simulink model "BLDCSpeedControl_EV_Layout_FINAL"  (R2024b)
settings: Solver=ode23t  StartTime=0.0  StopTime=t_stop  FixedStep=Ts  MaxStep=5e-4  RelTol=1e-3  EnableMultiTasking=on
PreLoadFcn:
  | BLDCSpeedControlData;
values from neighbouring files (symbols this model uses):
  m = app.Rows(1:app.N, 1) >= 0.9*t    [EV_BlackBox_App.m]
  N = 0    [EV_BlackBox_App.m]
  p = inputParser    [Create_Simulation.m]    (also in EV_BlackBox_App.m = uipanel(parent, 'Title', title); Run_Simulation_Live.m; Run_Simulation_Log.m)
  s = regexprep(msg, '\s+', ' ')    [EV_BlackBox_App.m]    (also in Run_Simulation_Log.m = T.SOC(isfinite(T.SOC)))
undefined symbols (not defined in the file or in its folder): battery_builder_rtmsupport, cells_parallel, cells_series, DiscIntNeverNeededParam, Emax, Emax_thr, emf_max_ev, gcbh, I_cont, I_peak, Ke_ph, Kii, Kiv, Kiw, Kpi, Kpv, Kpw, load_scale, r_wheel, rpm_ramp, rpm_ref, T_Ifilt, Ts, Tsc, Vdc, Vlim_min, wheel_mass
libraries: nesl_utility x19, fl_lib x13, ee_lib x6, sm_lib x3, eeDiscretePi x2, Batteries2_lib x1, SignalEditorBlockLib x1, eePwmGenerator x1, eeGeneralControl x1
(part 1 of 2)
CloseFcn:
  | try,close(h1_BLDCSpeedControl),end
  | clear h1_BLDCSpeedControl
  | 
  | clear simlog_BLDCSpeedControl
  | clear logsout_BLDCSpeedControl
Description:
  | BLDC Speed Control
settings Model: Creator=The MathWorks, Inc.  LastModifiedBy=shubh
settings SolverCC: AlgebraicLoopSolver=TrustRegion  MaxZcPerStep=1
settings DataIOCC: MaxDataPoints=210000  ReturnWorkspaceOutputs=off  SignalLoggingName=logsout_BLDCSpeedControl
settings OptimizationCC: ReuseModelBlockBuffer=off  LifeSpan=inf
settings DebuggingCC: UnconnectedInputMsg=warning  UnconnectedOutputMsg=warning  UnconnectedLineMsg=warning  SFUnexpectedBacktrackingDiag=warning  SFNoUnconditionalDefaultTransitionDiag=warning  SFExecutionAtInitializationDiag=none  ArithmeticOperatorsInVariantConditions=warning
settings ModelReferenceCC: EnableRefExpFcnMdlSchedulingChecks=on
settings SFSimCC: SimUseLocalCustomCode=off  CustomCodeUndefinedFunction=UseInterfaceOnly
settings RTWCC: RTWUseLocalCustomCode=off  GPUComputeCapability=3.5  DLArmComputeVersion=19.05
settings CodeAppCC: StateflowObjectComments=on
settings GRTTargetCC: TargetLangStandard=C89/C90 (ANSI)
settings ConfigComp: CovMetricSettings=dw  CovSaveCumulativeToWorkspaceVar=on  CovSaveSingleToWorkspaceVar=on  CovExternalEMLEnable=off
settings SimscapeCC: SimscapeNormalizeSystem=off  SimscapeLogSimulationStatistics=on  SimscapeLogName=simlog_BLDCSpeedControl  SimscapeLogLimitData=off  SimscapeLogDataHistory=210000
settings ExplorerConfigSet: SimMechanicsOpenEditorOnUpdate=off

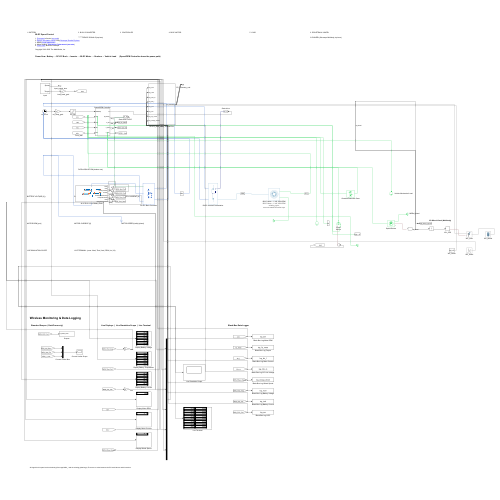
[thumbnail: Simulink's stored preview of the top-level diagram]
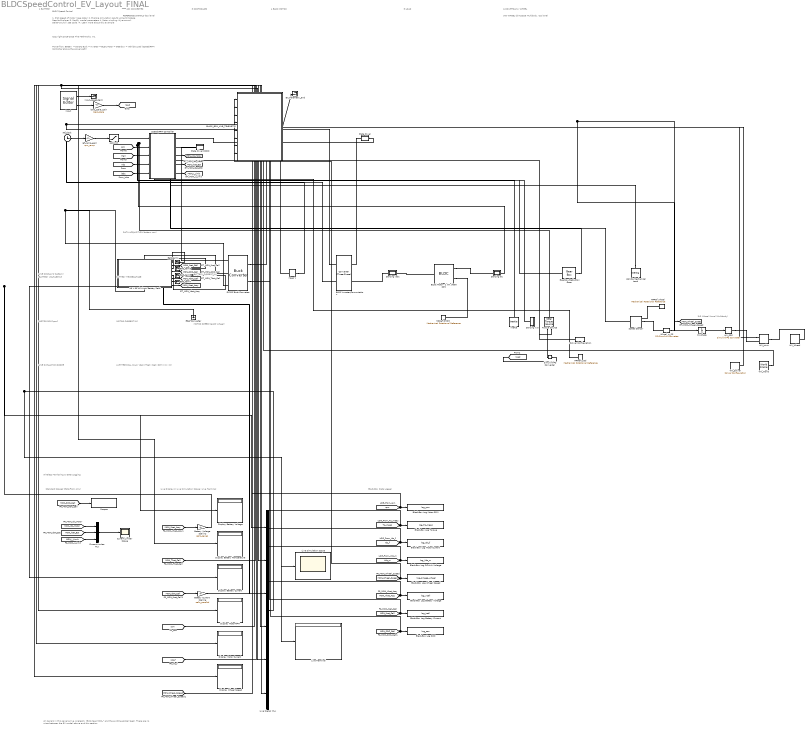
== system BLDCSpeedControl_EV_Layout_FINAL ==
  note: BLDC Speed Control
  note: 1. Plot speed of motor ( see code )
      | 2. Explore simulation results using Simscape Results Explorer
      | 3. Modify model parameters
      | 4. Motor winding: Wye-wound , Delta-wound ( see code )
      | 4. Learn more about this example
  note: Copyright 2016-2023 The MathWorks, Inc.
  note: BATTERY VOLTAGE [V]
  note: BATTERY TEMPERATURE
  note: BATTERY CURRENT [A]
  note: MOTOR RPM [rpm]
  note: MOTOR CURRENT [A]
  note: MOTOR SPEED [rad/s] (wheel)
  note: LIVE SIMULATION SCOPE
  note: LIVE TERMINAL (rows: Vbat | Tbat | Ibat | RPM | Im | W)
  note: 1 BATTERY
  note: 2 BUCK CONVERTER
  note: 3 CONTROLLER
  note: 4 BLDC MOTOR
  note: 5 LOAD
  note: 6 DRIVETRAIN / WHEEL
  note: REFERENCE SIGNALS (top lane)
  note: 3-D WHEEL (Simscape Multibody, top lane)
  note: DATA ACQUISITION (bottom row)
  note: LIVE DISPLAYS (bottom)
  note: Wireless Monitoring & Data Logging
  note: Standard Scopes (Goto/From only)
  note: Live Displays | Live Simulation Scope | Live Terminal
  note: Black-Box Data Logger
  note: All signals in this panel arrive wirelessly (Goto tags MON_* and the existing global tags). There are no wires between the EV model above and this section.
  note: Power flow: Battery → DC-DC Buck → Inverter → BLDC Motor → Gearbox → Vehicle Load (Speed/RPM Controller above the power path)
  note: 3-D Wheel Visual (Multibody)
  48 V 50 Ah Li-Ion Battery Pack : Subsystem  LoadFcn=battery_builder_rtmsupport('loadfcn',gcbh);
      settings: CopyFcn=battery_builder_rtmsupport('copyfcn',gcbh);  PreCopyFcn=battery_builder_rtmsupport('precopyfcn',gcbh);  PreDeleteFcn=battery_builder_rtmsupport('predeletefcn',gcbh);  PortSchema="{\"entries\":[{\"content\":{\"sides\":[{\"content\":{\"connectorIds\":[\"LConn1\"]},\"type\":\"ConnectorPlacement.EquallySpacedRectSide\",\"uuid\":\"bf691570-7ac9-499a-8942-6e8ffe2774e2\"},{\"content\":{\"connectorIds\":[\"RConn1\"],\"side\":\"RIGHT\"},\"type\":\"ConnectorPlacement.EquallySpacedRectSide\",\"uuid\":\"48e96f6a-2aee-45a9-a2ae-5a9441790c71\"},{\"content\":{\"side\":\"TOP\"},\"type\":\"ConnectorPlacement.EquallySpacedRectSide\",\"uuid\":\"dfdf2b0d-1e4b-464b-8a83-b0b25904b005\"},{\"content\":{\"connectorIds\":[\"Out1\",\"Out2\",\"Out3\",\"Out4\",\"Out5\",\"Out6\",\"Out7\",\"Out8\"],\"side\":\"BOTTOM\"},\"type\":\"ConnectorPlacement.EquallySpacedRectSide\",\"uuid\":\"0118fead-b379-4450-9723-57bbd90a7e7a\"}]},\"type\":\"ConnectorPlacement.EquallySpacedConnector\",\"uuid\":\"e9cae3f7-6351-471c-9be2-cb3ea8e3ac6a\"}],\"packageUris\":[\"http://schema.mathworks.com/mf0/Connector/R2020b\"],\"version\":\"1.0\"}"
      mask Display: image('$imagefile')
  BLACK_BOX_LIVE_TELEMETRY : Subsystem
  BLDC Inverter/Commutation : ee_lib/Semiconductors & Converters/Converters/Converter (Three-Phase)  port_option=ee.enum.threePhasePort.composite  fidelity_option=ee.enum.converters.fidelity.detailed  device_type=3  showThermalPort=false  K=0  Vth=0.5 V  Vgt=1 V  Vgt_off=-1 V  Ih=1 A  Vf=0.8 V  Ron=0.001 Ohm  Rds=0.001 Ohm  Goff=1e-5 1/Ohm  Eon_scalar=22.86e-3 J  Eoff_scalar=17.14e-3 J  Eoff_natural_commutation=10e-3 J  Voff=300 V  Iout_scalar=600 A  onCurrentMeasDelay=0 s  useCurrentFromPreviousCycle=false  useVoltageFromPreviousCycle=false  diode_param=2  diode_Vf=0.8 V  diode_Ron=0.001 Ohm  diode_Goff=1e-5 1/Ohm  diode_C=50 nF  diode_iRM=-235 A  diode_iF=300 A  diode_idot=-50 A/us  diode_trr_param=1  diode_trr_factor=3  diode_trr=15 us  diode_Qrr=1.5e+3 s*uA  diode_rec_loss_model=ee.enum.diode.reverseRecoveryModel.fixed  diode_ErecVal=0 J  diode_scaleWithIandV=false  diode_ErecMat=zeros(2, 3) J  diode_TjrecVec=[298.15, 398.15] K  diode_IfrecVec=[.1, 1, 10] A  diode_IrecVal=10 A  diode_VrecVal=10 V  diode_tFilter=1 / 1000 / 100 s  thermal_network_parameterization=ee.enum.thermalNetworkTopology.external  Rth=[.08, .5] K/W  Rth_Cauer=[.08, .1, .5] K/W  Rth_Foster=[.08, .14, .22, .16] K/W  thermal_mass_parameterization=ee.enum.thermalNetwork.timeconstant  thermal_mass=[.01, .5] J/K  thermal_mass_Cauer=[.01, .1, .5] J/K  thermal_mass_Foster=[.001, .005, .05, .5] J/K  thermal_time_constant=[.001, .2] s  thermal_time_constant_Cauer=[.001, .1, .2] s  thermal_time_constant_Foster=[7e-05, .0007, .01, .08] s  thermal_mass_initial_temperatures=[25, 25] degC  thermal_mass_initial_temperatures_Cauer=[25, 25, 25] degC  junction_thermal_mass=0.01 J/K  Tvec_initial_Foster=[25, 25, 25, 25] degC  snubber_type=0  Cs=1e-7 F  Rs=0.1 Ohm  Vce_loss=[0, 150, 300] V
  "BLDC Motor – 1 kW, 3000 RPM" : ee_lib/Electromechanical/Permanent Magnet/BLDC  port_option=ee.enum.threePhasePort.composite  rotor_param=1  pm_flux_linkage=psim Wb  theta_constant=pi / (2*p) rad  emf_max=emf_max_ev V  w_meas=w_meas_rpm rpm  DphiDtheta_tab=[0, -Ke_ph, -Ke_ph, Ke_ph, Ke_ph, 0] Wb/rad  back_emf_tab=[0, -emf_max_ev, -emf_max_ev, emf_max_ev, emf_max_ev, 0] V  rotor_angle_tab=[0, 7.5, 22.5, 37.5, 52.5, 60] deg  nPolePairs=p  axes_param=1  winding_type=ee.enum.statorconnection.wye  stator_param=2  machine_param=ee.enum.dqparameterization.constant  Ld=0.00022 H  Lq=0.00022 H  idVec=[-200, 0, 200] A  iqVec=[-200, 0, 200] A  LdMatrix=0.00022 * ones(3, 3) H  LqMatrix=0.00022 * ones(3, 3) H  L0=0.00016 H  Ls=Ls H  Lm=0 H  Ms=Ms H  Rs=Rs Ohm  zero_sequence=ee.enum.park.zerosequence.exclude  loss_param=ee.enum.ironloss.none  losses_oc=[0, 0, 0] W  losses_sc=[0, 0, 0] W  f_losses=60 Hz  Isc_losses=95 A  J=0 kg*m^2  lam=0 N*m/(rad/s)  i_d_specify=off  i_d_priority=None  i_d=0 A  i_d_nominal_specify=off  i_d_nominal_value=1  i_d_nominal_unit=A  i_q_specify=off  i_q_priority=None  i_q=0 A  i_q_nominal_specify=off  i_q_nominal_value=1  i_q_nominal_unit=A  torque_specify=off  torque_priority=None  torque=0 N*m  torque_nominal_specify=off  torque_nominal_value=1  torque_nominal_unit=N*m  angular_velocity_specify=off  angular_velocity_priority=High  angular_velocity=0 rpm  angular_velocity_nominal_specify=off  angular_velocity_nominal_value=1  angular_velocity_nominal_unit=rpm  angular_position_specify=off  angular_position_priority=High  angular_position=0 deg  angular_position_nominal_specify=off  angular_position_nominal_value=1  angular_position_nominal_unit=deg  alpha=3.93e-3 1/K  alpha_flux=-0.001 1/K  Tmeas=298.15 K  stator_thermal_mass=100 J/K  rotor_thermal_mass=200 J/K  Rm_percent_rotor=90  Rd_percent_rotor=30  temperatureA_specify=off  temperatureA_priority=High  temperatureA=25 degC  temperatureA_nominal_specify=off  temperatureA_nominal_value=1  temperatureA_nominal_unit=degC  temperatureB_specify=off  temperatureB_priority=High  temperatureB=25 degC  temperatureB_nominal_specify=off  temperatureB_nominal_value=1  temperatureB_nominal_unit=degC  temperatureC_specify=off  temperatureC_priority=High  temperatureC=25 degC  temperatureC_nominal_specify=off  temperatureC_nominal_value=1  temperatureC_nominal_unit=degC  temperatureR_specify=off  temperatureR_priority=High  temperatureR=25 degC  temperatureR_nominal_specify=off  temperatureR_nominal_value=1  temperatureR_nominal_unit=degC
      settings: InternalSimscapePortConfiguration="{\"Bottom\":[],\"Left\":[{\"id\":\"N\",\"label\":\"~\",\"type\":\"foundation.electrical.three_phase\"}],\"Right\":[{\"id\":\"R\",\"label\":\"R\",\"type\":\"foundation.mechanical.rotational.rotational\"},{\"id\":\"C\",\"label\":\"C\",\"type\":\"foundation.mechanical.rotational.rotational\"}],\"Top\":[]}"
      settings: AttributesFormatString=|
      | %<Name>
      | winding_type=
      | %<winding_type>
  Batt_term{1,3,5,7} (4 alike) : Terminator
  Battery Current Scaling : Gain  Gain=cells_parallel
  Battery Voltage Scaling : Gain  Gain=cells_series
  Black-Box Log Battery Current : ToWorkspace  VariableName=log_icell  SampleTime=-1
  Black-Box Log Battery Voltage : ToWorkspace  VariableName=log_vcell  SampleTime=-1
  Black-Box Log DC-Link Voltage : ToWorkspace  VariableName=log_Vdc_m  SampleTime=-1
  Black-Box Log Motor Current : ToWorkspace  VariableName=log_Idc_f  SampleTime=-1
  Black-Box Log Motor RPM : ToWorkspace  VariableName=log_rpm  SampleTime=-1
  Black-Box Log SOC : ToWorkspace  VariableName=log_soc  SampleTime=-1
  Black-Box Log Torque : ToWorkspace  VariableName=log_Tq_meas  SampleTime=-1
  Black-Box Log Wheel Speed : ToWorkspace  VariableName=log_omega_wheel  SampleTime=-1
  Current Limiter Mux : Mux  Inputs=3
  Current Limiter Scope : Scope
  DC-DC Buck Converter : ee_lib/Semiconductors & Converters/Converters/Buck Converter  port_option=ee.enum.controlport.ps  device_type=ee.enum.converters.switchingdevice.ideal  Vf=0.8 V  Ron=0.001 Ohm  Rds=0.001 Ohm  Goff=1e-5 1/Ohm  Vgt=1 V  Vgt_off=-1 V  Ih=1 A  Vth=0.5 V  K=0  diode_param=2  diode_Vf=0.8 V  diode_Ron=0.001 Ohm  diode_Goff=1e-5 1/Ohm  diode_C=50 nF  diode_iRM=-235 A  diode_iF=300 A  diode_idot=-50 A/us  diode_trr_param=1  diode_trr_factor=3  diode_trr=15 us  diode_Qrr=1500 s*uA  Lf=220 uH  Rl=0 Ohm  Cf=100 uF  Rf=.25 Ohm  snubber_type=1  Cs=1e-7 F  Rs=0.1 Ohm  iL_specify=off  iL_priority=High  iL=0 A  iL_nominal_specify=off  iL_nominal_value=1  iL_nominal_unit=A  vc_specify=off  vc_priority=High  vc=0 V  vc_nominal_specify=off  vc_nominal_value=1  vc_nominal_unit=V
      settings: InternalSimscapePortConfiguration="{\"Bottom\":[],\"Left\":[{\"id\":\"G\",\"label\":\"G\",\"type\":\"foundation.electrical.four_phase\"},{\"id\":\"p1\",\"label\":\"1+\",\"type\":\"foundation.electrical.electrical\"},{\"id\":\"n1\",\"label\":\"1-\",\"type\":\"foundation.electrical.electrical\"}],\"Right\":[{\"id\":\"p2\",\"label\":\"2+\",\"type\":\"foundation.electrical.electrical\"},{\"id\":\"n2\",\"label\":\"2-\",\"type\":\"foundation.electrical.electrical\"}],\"Top\":[]}"
  Display Battery Current : Display
  Display Battery Temperature : Display
  Display Battery Voltage : Display
  Display Motor Current : Display
  Display Motor RPM : Display
  Display Wheel Speed : Display
  ERef Converter : fl_lib/Electrical/Electrical Elements/Electrical Reference
  EV_Telemetry_end : Terminator
  Gate driver : Subsystem
  Gate driver DCDC : Subsystem
  Gearbox/Reduction Gear : fl_lib/Mechanical/Mechanisms/Gear Box  ratio=gear_ratio  t_in_specify=off  t_in_priority=None  t_in=0 N*m  t_in_nominal_specify=off  t_in_nominal_value=1  t_in_nominal_unit=N*m  t_out_specify=off  t_out_priority=None  t_out=0 N*m  t_out_nominal_specify=off  t_out_nominal_value=1  t_out_nominal_unit=N*m
  Inertia : fl_lib/Mechanical/Rotational Elements/Inertia  inertia="Jm  kg*m^2"  num_ports=foundation.enum.numPorts2.one  w_specify=on  w_priority=High  w=0 rpm  w_nominal_specify=off  w_nominal_value=1  w_nominal_unit=rad/s  t_specify=off  t_priority=High  t=0 N*m  t_nominal_specify=off  t_nominal_value=1  t_nominal_unit=N*m
  Input : SignalEditorBlockLib/Signal Editor  FileName=BLDCSpeedControlInput.mat  ActiveScenario=Test_1  ActiveSignal=Torque  IsBus=off  OutputBusObjectStr=Bus: BusObject  SampleTime=0  OutputAfterFinalValue=Extrapolation  Unit=inherit  PreserveSignalName=on  ApplySigPropsToAllScenarios=on  ApplySigPropsToAllSignals=off
  Input_speed_term : Terminator
  Live Signal Mux : Mux  Inputs=6
  Live Simulation Scope : Scope
  Live Terminal : Display
  MRRef IPMSM : fl_lib/Mechanical/Rotational Elements/Mechanical Rotational Reference
  MRRef Load : fl_lib/Mechanical/Rotational Elements/Mechanical Rotational Reference
  MRRef_wheel : fl_lib/Mechanical/Rotational Elements/Mechanical Rotational Reference
  Meas V : Subsystem
      mask Display: disp('Vdc')
  Scopes : Subsystem
  Sensing trq : Subsystem
      mask Display: disp('trq')
  Sensing w a : Subsystem
      mask Display: disp('w,Hall')
  Sensing iabc : Subsystem
      mask Display: disp('iabc')
  Simulink-PS Converter : nesl_utility/Simulink-PS Converter  PhysicalDomain=network_engine_domain  SubClassName=ps_input  LeftPortType=input  RightPortType=output  PseudoPeriodic=off  Frequencies=[]  NoiseDistribution=none  NoiseParameters=[]  Unit=N*m  AffineConversion=off  FilteringAndDerivatives=zero  SimscapeFilterOrder=1  InputFilterTimeConstant=0.001  UdotUserProvided=1
  Solver Configuration : nesl_utility/Solver Configuration  PhysicalDomain=network_engine_domain  SubClassName=solver  LeftPortType=input  RightPortType=generic  Tones=[]  Harmonics=[]  SimulateNoise=off  Profile=off  UseLocalSampling=off  EnableSwitchedLinearOptims=on  FrequencyDomain=off  UseCCode=off  RelTol=0.001  AbsTol=1e-06  MinStep=1e-09  ToWorkspace=off  RevertToSquareIcSolve=off  NumHomotopyIterations=100  PhasorMode=off  PhasorModeNumHarmonics=1  ConsistencySolver=NEWTON_FTOL  IndexReductionMethod=DerivativeReplacement  DoDC=off  ResidualTolerance=1e-9  ConsistencyTolSource=GLOBAL  ConsistencyAbsTol=0.001  ConsistencyRelTol=0.001  ConsistencyTolFactor=0.001  UseLocalSolver=on  LocalSolverChoice=NE_TRAPEZOIDAL_ADVANCER  ResolveIndetEquations=on  FunctionEvalNumThread=1  LocalSolverSampleTime=Ts  DoFixedCost=on  MaxNonlinIter=4  MaxModeIter=2  ComputeImpulses=off  ImpulseIterations=2  LinearAlgebra=auto  LinearAlgebraNumThread=0  EquationFormulation=NE_TIME_EF  DelaysMemoryBudget=1024  AutomaticFiltering=on  FilteringTimeConstant=0.001  PartitionStorageMethod=AS_NEEDED  PartitionMemoryBudget=1024  PartitionMethod=FAST  MultibodyUseLocalSolver=off  MultibodyLocalSolverChoice=ODE1  MultibodyLocalSolverSampleTime=0.001
  Speed Sensor : fl_lib/Mechanical/Mechanical Sensors/Ideal Rotational Motion Sensor  reference=foundation.enum.MeasurementReference.difference  acceleration_port=false  velocity_port=true  position_port=true  wrap_angle=false  offset=0 rad
  Speed/RPM Controller : Subsystem
  Torque Source : fl_lib/Mechanical/Mechanical Sources/Ideal Torque Source
  Vehicle Mechanical Load : fl_lib/Mechanical/Rotational Elements/Inertia  inertia=0.5*wheel_mass*r_wheel^2 kg*m^2  num_ports=foundation.enum.numPorts2.one  w_specify=off  w_priority=High  w=0 rad/s  w_nominal_specify=off  w_nominal_value=1  w_nominal_unit=rad/s  t_specify=off  t_priority=None  t=0 N*m  t_nominal_specify=off  t_nominal_value=1  t_nominal_unit=N*m
  WV_Joint : sm_lib/Joints/Revolute Joint  JointMode=Normal  CompositeWrenchDir=FollowerOnBase  CompositeWrenchFrame=BaseFrame  SenseConstraintForce=off  SenseConstraintTorque=off  SenseTotalForce=off  SenseTotalTorque=off  PositionTargetSpecify=off  PositionTargetPriority=High  PositionTargetValue=0  PositionTargetValueUnits=deg  VelocityTargetSpecify=off  VelocityTargetPriority=High  VelocityTargetValue=0  VelocityTargetValueUnits=deg/s  EquilibriumPosition=0  EquilibriumPositionUnits=deg  SpringStiffness=0  SpringStiffnessUnits=N*m/deg  DampingCoefficient=0  DampingCoefficientUnits=N*m/(deg/s)  LowerLimitSpecify=off  LowerLimitBound=-90  LowerLimitBoundUnits=deg  LowerLimitStiffness=1e4  LowerLimitStiffnessUnits=N*m/deg  LowerLimitDamping=10  LowerLimitDampingUnits=N*m/(deg/s)  LowerLimitTransitionRegionWidth=0.1  LowerLimitTransitionRegionWidthUnits=deg  UpperLimitSpecify=off  UpperLimitBound=90  UpperLimitBoundUnits=deg  UpperLimitStiffness=1e4  UpperLimitStiffnessUnits=N*m/deg  UpperLimitDamping=10  UpperLimitDampingUnits=N*m/(deg/s)  UpperLimitTransitionRegionWidth=0.1  UpperLimitTransitionRegionWidthUnits=deg  TorqueActuationMode=ComputedTorque  MotionActuationMode=InputMotion  SensePosition=off  SenseVelocity=off  SenseAcceleration=off  SenseTorqueForce=off  SenseLowerLimitTorqueForce=off  SenseUpperLimitTorqueForce=off
  WV_SPS : nesl_utility/Simulink-PS Converter  PhysicalDomain=network_engine_domain  SubClassName=ps_input  LeftPortType=input  RightPortType=output  PseudoPeriodic=off  Frequencies=[]  NoiseDistribution=none  NoiseParameters=[]  Unit=1  AffineConversion=off  FilteringAndDerivatives=filter  SimscapeFilterOrder=2  InputFilterTimeConstant=0.001  UdotUserProvided=0
  WV_Solver : nesl_utility/Solver Configuration  PhysicalDomain=network_engine_domain  SubClassName=solver  LeftPortType=input  RightPortType=generic  Tones=[]  Harmonics=[]  SimulateNoise=off  Profile=off  UseLocalSampling=off  EnableSwitchedLinearOptims=on  FrequencyDomain=off  UseCCode=off  RelTol=0.001  AbsTol=0.001  MinStep=1e-09  ToWorkspace=off  RevertToSquareIcSolve=off  NumHomotopyIterations=100  PhasorMode=off  PhasorModeNumHarmonics=1  ConsistencySolver=NEWTON_XTOL_AFTER_FTOL  IndexReductionMethod=DerivativeReplacement  DoDC=off  ResidualTolerance=1e-09  ConsistencyTolSource=GLOBAL  ConsistencyAbsTol=0.001  ConsistencyRelTol=0.001  ConsistencyTolFactor=0.001  UseLocalSolver=off  LocalSolverChoice=NE_BACKWARD_EULER_ADVANCER  ResolveIndetEquations=on  FunctionEvalNumThread=1  LocalSolverSampleTime=0.001  DoFixedCost=off  MaxNonlinIter=3  MaxModeIter=2  ComputeImpulses=off  ImpulseIterations=2  LinearAlgebra=auto  LinearAlgebraNumThread=0  EquationFormulation=NE_TIME_EF  DelaysMemoryBudget=1024  AutomaticFiltering=on  FilteringTimeConstant=0.001  PartitionStorageMethod=AS_NEEDED  PartitionMemoryBudget=1024  PartitionMethod=ROBUST  MultibodyUseLocalSolver=off  MultibodyLocalSolverChoice=ODE1  MultibodyLocalSolverSampleTime=0.001
  WV_Wheel : sm_lib/Body Elements/Cylindrical Solid  CylinderRadius=r_wheel  CylinderRadiusUnits=m  CylinderLength=wheel_width  CylinderLengthUnits=m  ExportEntireGeometry=off  InertiaType=CalculateFromGeometry  BasedOnType=Mass  Density=1000  DensityUnits=kg/m^3  Mass=wheel_mass  MassUnits=kg  CenterOfMass=[0 0 0]  CenterOfMassUnits=m  MomentsOfInertia=[1 1 1]  MomentsOfInertiaUnits=kg*m^2  ProductsOfInertia=[0 0 0]  ProductsOfInertiaUnits=kg*m^2  GraphicType=FromGeometry  MarkerShape=Sphere  MarkerSize=10  GraphicVisPropType=SimpleVisualProperties  GraphicDiffuseColor=[0.5 0.5 0.5]  GraphicOpacity=1  GraphicSpecularColor=[0.5 0.5 0.5 1.0]  GraphicAmbientColor=[0.15 0.15 0.15 1.0]  GraphicEmissiveColor=[0.0 0.0 0.0 1.0]  GraphicShininess=75  DoExposeReferenceFrame=on  SerializedFrames=<Frames/>
  WV_World : sm_lib/Frames and Transforms/World Frame
  WV_theta : Integrator
  Wheel_w_PS : nesl_utility/PS-Simulink Converter  PhysicalDomain=network_engine_domain  SubClassName=ps_output  LeftPortType=input  RightPortType=output  PseudoPeriodic=off  Frequencies=[]  VectorFormat=inherit  Unit=rad/s  AffineConversion=off
  load_scale_gain : Gain  Gain=load_scale
  ref_clock : Clock
  ref_limit : Saturate  UpperLimit=rpm_ref  LowerLimit=0
  ref_ramp_gain : Gain  Gain=rpm_ramp
  tag scope: MON_I_Limit=global, MON_Ibat_Cell=global, MON_Ibat_Est=global, MON_Idc_Motor=global, MON_SOC_Cell=global, MON_Tbat_Cell=global, MON_Vbat_Assy=global, MON_Wheel_Speed=global, load=global
  wires:
  Speed/RPM Controller/1(S) -> Gate driver/1(S)
  [rpm] -> Speed/RPM Controller/2(rpm)
  [Hall] -> Speed/RPM Controller/3(Hall)
  Speed/RPM Controller/2(S_DCDC) -> Gate driver DCDC/1(S)  "Idc_f"
  [Vdc] -> Speed/RPM Controller/4(Vdc)
  [load] -> Simulink-PS Converter/1
  48 V 50 Ah Li-Ion Battery Pack/1(socOutCell) -> Batt_term1/1
  48 V 50 Ah Li-Ion Battery Pack/3(numCyclesCell) -> Batt_term3/1
  48 V 50 Ah Li-Ion Battery Pack/5(socParallelAssembly) -> Batt_term5/1
  48 V 50 Ah Li-Ion Battery Pack/7(vCell) -> Batt_term7/1
  Input/1 -> Input_speed_term/1
  ref_clock/1 -> ref_ramp_gain/1
  ref_ramp_gain/1 -> ref_limit/1
  ref_limit/1 -> Speed/RPM Controller/1(RPMReq)
  Input/2 -> load_scale_gain/1
  load_scale_gain/1 -> [load]
  [iabc] -> Speed/RPM Controller/5(iabc)
  WV_theta/1 -> WV_SPS/1
  Current Limiter Mux/1 -> Current Limiter Scope/1
  [Tq_meas] -> Black-Box Log Torque/1, BLACK_BOX_LIVE_TELEMETRY/7(log_Tq_meas)
  [Vdc_m] -> Black-Box Log DC-Link Voltage/1, BLACK_BOX_LIVE_TELEMETRY/3(log_Vdc_m)
  Battery Voltage Scaling/1 -> Display Battery Voltage/1, Live Signal Mux/1  "Vbat"
  Battery Current Scaling/1 -> Display Battery Current/1, Live Signal Mux/3  "Ibat"
  Live Signal Mux/1 -> Live Simulation Scope/1, Live Terminal/1
  48 V 50 Ah Li-Ion Battery Pack/4(socCell) -> [MON_SOC_Cell]  "socCell"
  [MON_SOC_Cell] -> Scopes/1(in_BATT_SOC)
  [MON_SOC_Cell] -> Black-Box Log SOC/1, BLACK_BOX_LIVE_TELEMETRY/6(log_soc)
  48 V 50 Ah Li-Ion Battery Pack/8(vParallelAssembly) -> [MON_Vbat_Assy]  "vAssy"
  [MON_Vbat_Assy] -> Black-Box Log Battery Voltage/1, BLACK_BOX_LIVE_TELEMETRY/2(log_vcell)
  [MON_Vbat_Assy] -> Battery Voltage Scaling/1
  48 V 50 Ah Li-Ion Battery Pack/2(iCell) -> [MON_Ibat_Cell]  "iCell"
  [MON_Ibat_Cell] -> Black-Box Log Battery Current/1, BLACK_BOX_LIVE_TELEMETRY/1(log_icell)
  [MON_Ibat_Cell] -> Battery Current Scaling/1
  48 V 50 Ah Li-Ion Battery Pack/6(temperatureCell) -> [MON_Tbat_Cell]  "tCell"
  [MON_Tbat_Cell] -> Display Battery Temperature/1, Live Signal Mux/2
  Wheel_w_PS/1 -> WV_theta/1, [MON_Wheel_Speed]  "w_wheel"
  [MON_Wheel_Speed] -> Black-Box Log Wheel Speed/1, BLACK_BOX_LIVE_TELEMETRY/8(log_omega_wheel)
  [MON_Wheel_Speed] -> Display Wheel Speed/1, Live Signal Mux/6
  Speed/RPM Controller/3(o_Idc) -> [MON_Idc_Motor]  "Ibat_est"
  [MON_Idc_Motor] -> Current Limiter Mux/1
  Speed/RPM Controller/4(o_Ibat) -> [MON_Ibat_Est]  "I_lim"
  [MON_Ibat_Est] -> Current Limiter Mux/2
  Speed/RPM Controller/5(o_Ilim) -> [MON_I_Limit]
  [MON_I_Limit] -> Current Limiter Mux/3
  [rpm] -> Black-Box Log Motor RPM/1, BLACK_BOX_LIVE_TELEMETRY/5(log_rpm)
  [rpm] -> Display Motor RPM/1, Live Signal Mux/4
  [Idc_f] -> Black-Box Log Motor Current/1, BLACK_BOX_LIVE_TELEMETRY/4(log_Idc_f)
  [Idc_f] -> Display Motor Current/1, Live Signal Mux/5
  BLACK_BOX_LIVE_TELEMETRY/1(EV_Telemetry) -> EV_Telemetry_end/1
  connections:
  DC-DC Buck Converter/RConn1 -- Meas V/LConn1 -- BLDC Inverter/Commutation/RConn1
  Torque Source/LConn1 -- Sensing trq/RConn1 -- Inertia/LConn1 -- Gearbox/Reduction Gear/LConn1 -- Sensing w a/LConn1
  Gate driver/RConn1 -- BLDC Inverter/Commutation/LConn1
  Torque Source/RConn1 -- Simulink-PS Converter/RConn1
  Torque Source/RConn2 -- Solver Configuration/RConn1 -- MRRef Load/LConn1
  Sensing iabc/LConn1 -- BLDC Inverter/Commutation/LConn2
  "BLDC Motor – 1 kW, 3000 RPM"/LConn1 -- Sensing iabc/RConn1
  "BLDC Motor – 1 kW, 3000 RPM"/RConn2 -- MRRef IPMSM/LConn1
  "BLDC Motor – 1 kW, 3000 RPM"/RConn1 -- Sensing trq/LConn1
  DC-DC Buck Converter/RConn2 -- Meas V/RConn1 -- BLDC Inverter/Commutation/RConn2
  Gate driver DCDC/RConn1 -- DC-DC Buck Converter/LConn1
  48 V 50 Ah Li-Ion Battery Pack/LConn1 -- DC-DC Buck Converter/LConn2
  DC-DC Buck Converter/LConn3 -- 48 V 50 Ah Li-Ion Battery Pack/RConn1 -- ERef Converter/LConn1
  Vehicle Mechanical Load/LConn1 -- Gearbox/Reduction Gear/RConn1 -- Speed Sensor/LConn1
  MRRef_wheel/LConn1 -- Speed Sensor/RConn1
  Speed Sensor/RConn2 -- Wheel_w_PS/LConn1
  WV_Joint/LConn1 -- WV_World/RConn1 -- WV_Solver/RConn1
  WV_SPS/RConn1 -- WV_Joint/LConn2
  WV_Joint/RConn1 -- WV_Wheel/RConn1

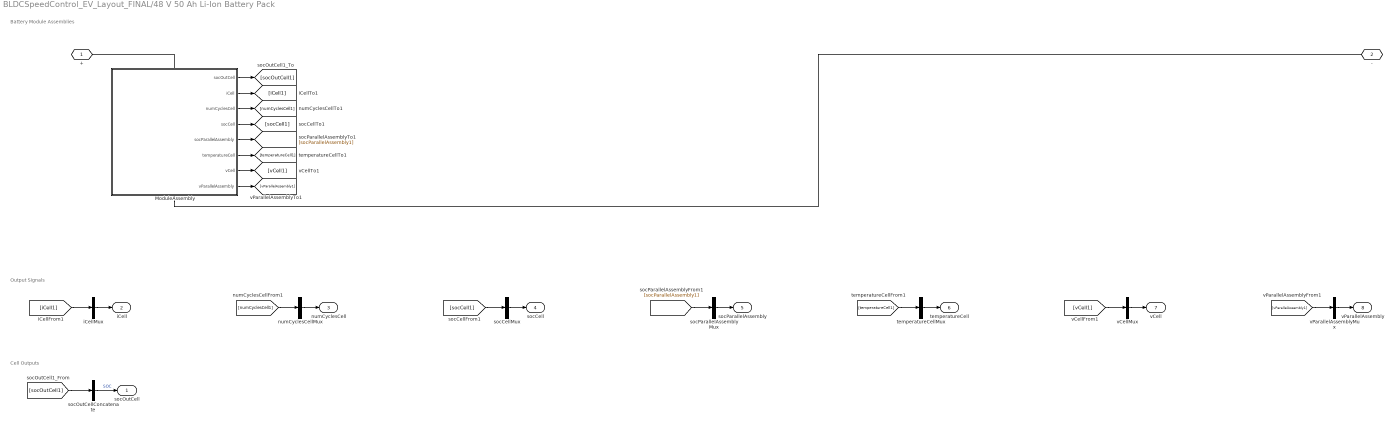
== system BLDCSpeedControl_EV_Layout_FINAL/48 V 50 Ah Li-Ion Battery Pack ==
  note: Cell Outputs
  note: Output Signals
  note: Battery Module Assemblies
  ModuleAssembly : Subsystem  LoadFcn=battery_builder_rtmsupport('loadfcn',gcbh);
      settings: CopyFcn=battery_builder_rtmsupport('copyfcn',gcbh);  PreCopyFcn=battery_builder_rtmsupport('precopyfcn',gcbh);  PreDeleteFcn=battery_builder_rtmsupport('predeletefcn',gcbh);  PortSchema="{\"entries\":[{\"content\":{\"sides\":[{\"content\":{\"connectorIds\":[\"LConn1\"]},\"type\":\"ConnectorPlacement.EquallySpacedRectSide\",\"uuid\":\"bf691570-7ac9-499a-8942-6e8ffe2774e2\"},{\"content\":{\"connectorIds\":[\"RConn1\"],\"side\":\"RIGHT\"},\"type\":\"ConnectorPlacement.EquallySpacedRectSide\",\"uuid\":\"48e96f6a-2aee-45a9-a2ae-5a9441790c71\"},{\"content\":{\"side\":\"TOP\"},\"type\":\"ConnectorPlacement.EquallySpacedRectSide\",\"uuid\":\"dfdf2b0d-1e4b-464b-8a83-b0b25904b005\"},{\"content\":{\"connectorIds\":[\"Out1\",\"Out2\",\"Out3\",\"Out4\",\"Out5\",\"Out6\",\"Out7\",\"Out8\"],\"side\":\"BOTTOM\"},\"type\":\"ConnectorPlacement.EquallySpacedRectSide\",\"uuid\":\"4677a5a2-4e77-4e4b-9685-54aec05e9f00\"}]},\"type\":\"ConnectorPlacement.EquallySpacedConnector\",\"uuid\":\"e9cae3f7-6351-471c-9be2-cb3ea8e3ac6a\"}],\"packageUris\":[\"http://schema.mathworks.com/mf0/Connector/R2020b\"],\"version\":\"1.0\"}"
      mask Display: image('$imagefile')
  iCellMux : Mux  Inputs=1
  numCyclesCellMux : Mux  Inputs=1
  socCellMux : Mux  Inputs=1
  socOutCellConcatenate : Concatenate  NumInputs=1  Mode=Multidimensional array  ConcatenateDimension=2
  socParallelAssemblyMux : Mux  Inputs=1
  temperatureCellMux : Mux  Inputs=1
  vCellMux : Mux  Inputs=1
  vParallelAssemblyMux : Mux  Inputs=1
  + : PMIOPort  Side=Left
  - : PMIOPort  Port=2  Side=Right
  socOutCell : Outport
  iCell : Outport  Port=2
  numCyclesCell : Outport  Port=3
  socCell : Outport  Port=4
  socParallelAssembly : Outport  Port=5
  temperatureCell : Outport  Port=6
  vCell : Outport  Port=7
  vParallelAssembly : Outport  Port=8
  wires:
  ModuleAssembly/1(socOutCell) -> [socOutCell1]
  [vParallelAssembly1] -> vParallelAssemblyMux/1
  vParallelAssemblyMux/1 -> vParallelAssembly/1
  ModuleAssembly/8(vParallelAssembly) -> [vParallelAssembly1]
  [vCell1] -> vCellMux/1
  vCellMux/1 -> vCell/1
  ModuleAssembly/7(vCell) -> [vCell1]
  [temperatureCell1] -> temperatureCellMux/1
  temperatureCellMux/1 -> temperatureCell/1
  ModuleAssembly/6(temperatureCell) -> [temperatureCell1]
  [socParallelAssembly1] -> socParallelAssemblyMux/1
  socParallelAssemblyMux/1 -> socParallelAssembly/1
  ModuleAssembly/5(socParallelAssembly) -> [socParallelAssembly1]
  [socCell1] -> socCellMux/1
  socCellMux/1 -> socCell/1
  ModuleAssembly/4(socCell) -> [socCell1]
  [numCyclesCell1] -> numCyclesCellMux/1
  numCyclesCellMux/1 -> numCyclesCell/1
  ModuleAssembly/3(numCyclesCell) -> [numCyclesCell1]
  [iCell1] -> iCellMux/1
  iCellMux/1 -> iCell/1
  ModuleAssembly/2(iCell) -> [iCell1]
  [socOutCell1] -> socOutCellConcatenate/1
  socOutCellConcatenate/1 -> socOutCell/1  "SOC"
  connections:
  ModuleAssembly/RConn1 -- -/RConn1
  ModuleAssembly/LConn1 -- +/RConn1

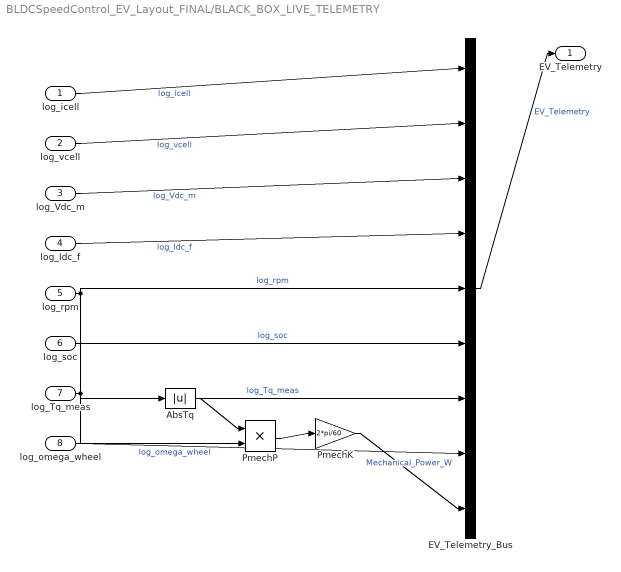
== system BLDCSpeedControl_EV_Layout_FINAL/BLACK_BOX_LIVE_TELEMETRY ==
  log_icell : Inport
  log_vcell : Inport  Port=2
  log_Vdc_m : Inport  Port=3
  log_Idc_f : Inport  Port=4
  log_rpm : Inport  Port=5
  log_soc : Inport  Port=6
  log_Tq_meas : Inport  Port=7
  log_omega_wheel : Inport  Port=8
  AbsTq : Abs  SaturateOnIntegerOverflow=off
  EV_Telemetry_Bus : BusCreator  Inputs=9
  PmechK : Gain  Gain=2*pi/60
  PmechP : Product
  EV_Telemetry : Outport
  wires:
  log_icell/1 -> EV_Telemetry_Bus/1  "log_icell"
  log_vcell/1 -> EV_Telemetry_Bus/2  "log_vcell"
  log_Vdc_m/1 -> EV_Telemetry_Bus/3  "log_Vdc_m"
  log_Idc_f/1 -> EV_Telemetry_Bus/4  "log_Idc_f"
  log_rpm/1 -> EV_Telemetry_Bus/5, PmechP/2  "log_rpm"
  log_soc/1 -> EV_Telemetry_Bus/6  "log_soc"
  log_Tq_meas/1 -> EV_Telemetry_Bus/7, AbsTq/1  "log_Tq_meas"
  log_omega_wheel/1 -> EV_Telemetry_Bus/8  "log_omega_wheel"
  AbsTq/1 -> PmechP/1
  PmechP/1 -> PmechK/1
  PmechK/1 -> EV_Telemetry_Bus/9  "Mechanical_Power_W"
  EV_Telemetry_Bus/1 -> EV_Telemetry/1  "EV_Telemetry"

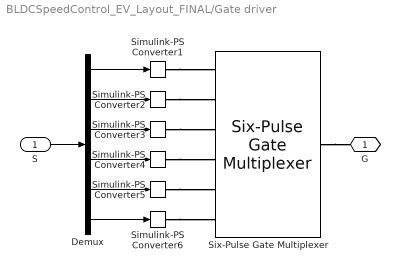
== system BLDCSpeedControl_EV_Layout_FINAL/Gate driver ==
  S : Inport
  Demux : Demux  Outputs=6
  Simulink-PS Converter{1..6} (6 alike) : nesl_utility/Simulink-PS Converter  PhysicalDomain=network_engine_domain  SubClassName=ps_input  LeftPortType=input  RightPortType=output  PseudoPeriodic=off  Frequencies=[]  NoiseDistribution=none  NoiseParameters=[]  Unit=1  AffineConversion=off  FilteringAndDerivatives=zero  SimscapeFilterOrder=1  InputFilterTimeConstant=0.001  UdotUserProvided=1
  Six-Pulse Gate Multiplexer : ee_lib/Semiconductors & Converters/Converters/Six-Pulse Gate Multiplexer  port_option=ee.enum.controlport.ps
  G : PMIOPort  Side=Right
  wires:
  Demux/1 -> Simulink-PS Converter1/1
  S/1 -> Demux/1
  Demux/4 -> Simulink-PS Converter4/1
  Demux/2 -> Simulink-PS Converter2/1
  Demux/3 -> Simulink-PS Converter3/1
  Demux/5 -> Simulink-PS Converter5/1
  Demux/6 -> Simulink-PS Converter6/1
  connections:
  Six-Pulse Gate Multiplexer/RConn1 -- G/RConn1
  Simulink-PS Converter1/RConn1 -- Six-Pulse Gate Multiplexer/LConn1
  Simulink-PS Converter3/RConn1 -- Six-Pulse Gate Multiplexer/LConn3
  Simulink-PS Converter5/RConn1 -- Six-Pulse Gate Multiplexer/LConn5
  Simulink-PS Converter6/RConn1 -- Six-Pulse Gate Multiplexer/LConn6
  Simulink-PS Converter4/RConn1 -- Six-Pulse Gate Multiplexer/LConn4
  Simulink-PS Converter2/RConn1 -- Six-Pulse Gate Multiplexer/LConn2

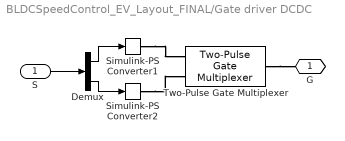
== system BLDCSpeedControl_EV_Layout_FINAL/Gate driver DCDC ==
  S : Inport
  Demux : Demux  Outputs=2
  Simulink-PS Converter1 : nesl_utility/Simulink-PS Converter  PhysicalDomain=network_engine_domain  SubClassName=ps_input  LeftPortType=input  RightPortType=output  PseudoPeriodic=off  Frequencies=[]  NoiseDistribution=none  NoiseParameters=[]  Unit=V  AffineConversion=off  FilteringAndDerivatives=zero  SimscapeFilterOrder=1  InputFilterTimeConstant=0.001  UdotUserProvided=1
  Simulink-PS Converter2 : nesl_utility/Simulink-PS Converter  PhysicalDomain=network_engine_domain  SubClassName=ps_input  LeftPortType=input  RightPortType=output  PseudoPeriodic=off  Frequencies=[]  NoiseDistribution=none  NoiseParameters=[]  Unit=V  AffineConversion=off  FilteringAndDerivatives=zero  SimscapeFilterOrder=1  InputFilterTimeConstant=0.001  UdotUserProvided=1
  Two-Pulse Gate Multiplexer : ee_lib/Semiconductors & Converters/Converters/Two-Pulse Gate Multiplexer  port_option=ee.enum.controlport.ps
      settings: InternalSimscapePortConfiguration="{\"Bottom\":[],\"Left\":[{\"id\":\"G1_ps\",\"label\":\"G1\",\"type\":\"input\"},{\"id\":\"G2_ps\",\"label\":\"G2\",\"type\":\"input\"}],\"Right\":[{\"id\":\"p\",\"label\":\"G\",\"type\":\"foundation.electrical.four_phase\"}],\"Top\":[]}"
  G : PMIOPort  Side=Right
  wires:
  Demux/1 -> Simulink-PS Converter1/1
  Demux/2 -> Simulink-PS Converter2/1
  S/1 -> Demux/1
  connections:
  Two-Pulse Gate Multiplexer/RConn1 -- G/RConn1
  Simulink-PS Converter1/RConn1 -- Two-Pulse Gate Multiplexer/LConn1
  Simulink-PS Converter2/RConn1 -- Two-Pulse Gate Multiplexer/LConn2

== system BLDCSpeedControl_EV_Layout_FINAL/Meas V ==
  PS-Simulink Converter2 : nesl_utility/PS-Simulink Converter  PhysicalDomain=network_engine_domain  SubClassName=ps_output  LeftPortType=input  RightPortType=output  PseudoPeriodic=off  Frequencies=[]  VectorFormat=1-D array  Unit=V  AffineConversion=off
  Voltage Sensor : fl_lib/Electrical/Electrical Sensors/Voltage Sensor
  + : PMIOPort  Side=Left
  - : PMIOPort  Port=2  Side=Right
  tag scope: Vdc=global
  wires:
  PS-Simulink Converter2/1 -> [Vdc]
  connections:
  Voltage Sensor/LConn1 -- +/RConn1
  PS-Simulink Converter2/LConn1 -- Voltage Sensor/RConn1
  Voltage Sensor/RConn2 -- -/RConn1

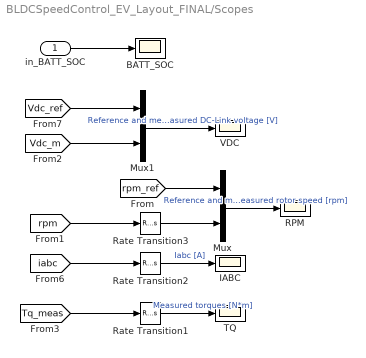
== system BLDCSpeedControl_EV_Layout_FINAL/Scopes ==
  in_BATT_SOC : Inport
  BATT_SOC : Scope
  IABC : Scope
  Mux : Mux  Inputs=2
  Mux1 : Mux  Inputs=2
  RPM : Scope
  Rate Transition1 : RateTransition
  Rate Transition2 : RateTransition  OutPortSampleTime=1e-4
  Rate Transition3 : RateTransition
  TQ : Scope
  VDC : Scope
  wires:
  in_BATT_SOC/1 -> BATT_SOC/1
  [Tq_meas] -> Rate Transition1/1
  Mux1/1 -> VDC/1  "Reference and measured DC-Link voltage [V]"
  [iabc] -> Rate Transition2/1
  Mux/1 -> RPM/1  "Reference and measured rotor speed [rpm]"
  [Vdc_ref] -> Mux1/1
  [rpm] -> Rate Transition3/1
  [Vdc_m] -> Mux1/2
  [rpm_ref] -> Mux/1
  Rate Transition3/1 -> Mux/2
  Rate Transition2/1 -> IABC/1  "Iabc [A]"
  Rate Transition1/1 -> TQ/1  "Measured torques [N*m]"

== system BLDCSpeedControl_EV_Layout_FINAL/Sensing trq ==
  PS-Simulink Converter3 : nesl_utility/PS-Simulink Converter  PhysicalDomain=network_engine_domain  SubClassName=ps_output  LeftPortType=input  RightPortType=output  PseudoPeriodic=off  Frequencies=[]  VectorFormat=1-D array  Unit=N*m  AffineConversion=off
  Torque Sensor : fl_lib/Mechanical/Mechanical Sensors/Ideal Torque Sensor
  R : PMIOPort  Side=Left
  C : PMIOPort  Port=2  Side=Right
  tag scope: Tq_meas=global
  wires:
  PS-Simulink Converter3/1 -> [Tq_meas]
  connections:
  Torque Sensor/RConn1 -- C/RConn1
  Torque Sensor/RConn2 -- PS-Simulink Converter3/LConn1
  Torque Sensor/LConn1 -- R/RConn1

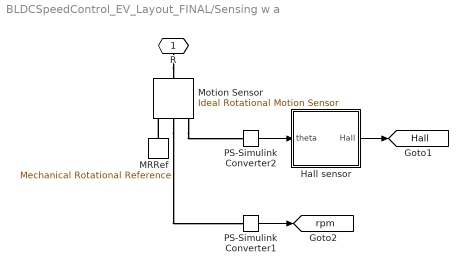
== system BLDCSpeedControl_EV_Layout_FINAL/Sensing w a ==
  Hall sensor : Subsystem
  MRRef : fl_lib/Mechanical/Rotational Elements/Mechanical Rotational Reference
  Motion Sensor : fl_lib/Mechanical/Mechanical Sensors/Ideal Rotational Motion Sensor  reference=foundation.enum.MeasurementReference.difference  acceleration_port=false  velocity_port=true  position_port=true  wrap_angle=simscape.enum.onoff.off  offset=0 deg
  PS-Simulink Converter1 : nesl_utility/PS-Simulink Converter  PhysicalDomain=network_engine_domain  SubClassName=ps_output  LeftPortType=input  RightPortType=output  PseudoPeriodic=off  Frequencies=[]  VectorFormat=1-D array  Unit=rpm  AffineConversion=off
  PS-Simulink Converter2 : nesl_utility/PS-Simulink Converter  PhysicalDomain=network_engine_domain  SubClassName=ps_output  LeftPortType=input  RightPortType=output  PseudoPeriodic=off  Frequencies=[]  VectorFormat=1-D array  Unit=rad  AffineConversion=off
  R : PMIOPort  Side=Left
  tag scope: Hall=global, rpm=global
  wires:
  PS-Simulink Converter1/1 -> [rpm]
  PS-Simulink Converter2/1 -> Hall sensor/1(theta)
  Hall sensor/1(Hall) -> [Hall]
  connections:
  R/RConn1 -- Motion Sensor/LConn1
  Motion Sensor/RConn2 -- PS-Simulink Converter1/LConn1
  MRRef/LConn1 -- Motion Sensor/RConn1
  Motion Sensor/RConn3 -- PS-Simulink Converter2/LConn1

== system BLDCSpeedControl_EV_Layout_FINAL/Sensing iabc ==
  Current Sensor : ee_lib/Sensors & Transducers/Current Sensor (Three-Phase)
  PS-Simulink Converter : nesl_utility/PS-Simulink Converter  PhysicalDomain=network_engine_domain  SubClassName=ps_output  LeftPortType=input  RightPortType=output  PseudoPeriodic=off  Frequencies=[]  VectorFormat=1-D array  Unit=A  AffineConversion=off
  1 : PMIOPort  Side=Left
  2 : PMIOPort  Port=2  Side=Right
  tag scope: iabc=global
  wires:
  PS-Simulink Converter/1 -> [iabc]
  connections:
  1/RConn1 -- Current Sensor/LConn1
  2/RConn1 -- Current Sensor/RConn2
  Current Sensor/RConn1 -- PS-Simulink Converter/LConn1

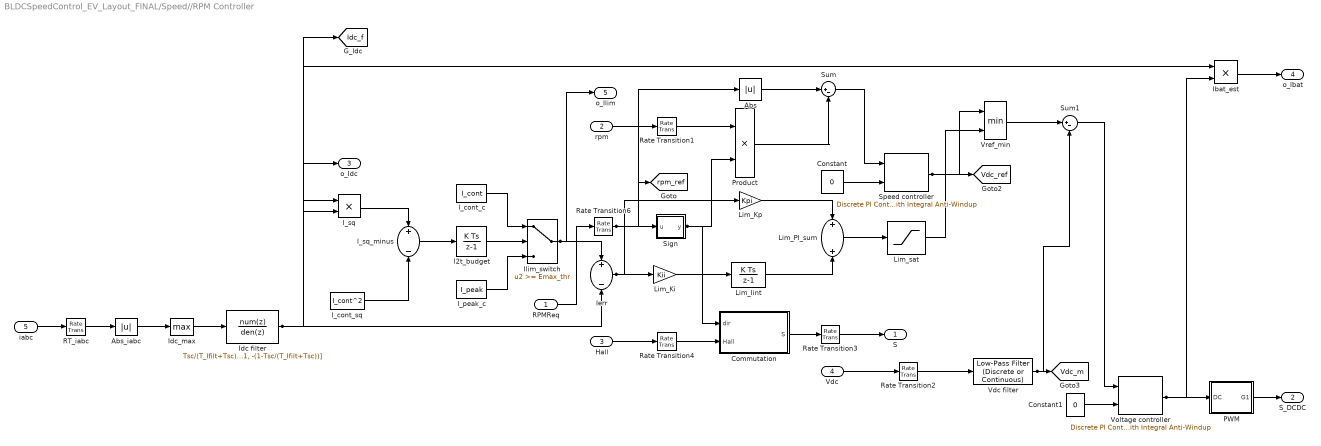
== system BLDCSpeedControl_EV_Layout_FINAL/Speed//RPM Controller ==
  RPMReq : Inport
  rpm : Inport  Port=2
  Hall : Inport  Port=3
  Vdc : Inport  Port=4
  iabc : Inport  Port=5
  Abs : Abs  SaturateOnIntegerOverflow=off
  Abs_iabc : Abs  SaturateOnIntegerOverflow=off
  Commutation : Subsystem
  Constant : Constant  Value=0  SampleTime=Tsc
  Constant1 : Constant  Value=0  SampleTime=Tsc
  I2t_budget : DiscreteIntegrator  SampleTime=Tsc  LimitOutput=on  UpperSaturationLimit=Emax  LowerSaturationLimit=0  ICPrevOutput=DiscIntNeverNeededParam  ICPrevScaledInput=DiscIntNeverNeededParam
  I_cont_c : Constant  Value=I_cont
  I_cont_sq : Constant  Value=I_cont^2
  I_peak_c : Constant  Value=I_peak
  I_sq : Product
  I_sq_minus : Sum  Inputs=+-
  Ibat_est : Product
  Idc filter : DiscreteTransferFcn  Numerator=Tsc/(T_Ifilt+Tsc)  Denominator=[1, -(1-Tsc/(T_Ifilt+Tsc))]  SampleTime=Tsc
  Idc_max : MinMax  Function=max
  Ierr : Sum  Inputs=+-
  Ilim_switch : Switch  Threshold=Emax_thr  SaturateOnIntegerOverflow=off  InputSameDT=off
  Lim_Iint : DiscreteIntegrator  InitialCondition=Vlim_min  SampleTime=Tsc  LimitOutput=on  UpperSaturationLimit=Vdc  LowerSaturationLimit=Vlim_min  ICPrevOutput=DiscIntNeverNeededParam  ICPrevScaledInput=DiscIntNeverNeededParam
  Lim_Ki : Gain  Gain=Kii
  Lim_Kp : Gain  Gain=Kpi
  Lim_PI_sum : Sum
  Lim_sat : Saturate  UpperLimit=Vdc  LowerLimit=Vlim_min
  PWM : Subsystem
  Product : Product
  RT_iabc : RateTransition
  Rate Transition1 : RateTransition
  Rate Transition2 : RateTransition
  Rate Transition3 : RateTransition  OutPortSampleTime=Ts
  Rate Transition4 : RateTransition  OutPortSampleTime=Tsc
  Rate Transition6 : RateTransition
  Sign : Subsystem
  Speed controller : eeDiscretePi/Discrete PI Controller with Integral Anti-Windup  Kp=Kpw  Ki=Kiw  x0=0  B=Vdc  A=0  Ts=Tsc
  Sum : Sum  Inputs=|+-
  Sum1 : Sum  Inputs=|+-
  Vdc filter : eeGeneralControl/Low-Pass Filter (Discrete or Continuous)  K=1  T=0.01  B=inf  A=-inf  init_option=Inherited from block input  x0=0  Ts=Tsc
  Voltage controller : eeDiscretePi/Discrete PI Controller with Integral Anti-Windup  Kp=Kpv  Ki=Kiv  x0=0  B=1  A=0  Ts=Tsc
  Vref_min : MinMax  Inputs=2
  S : Outport  VectorParamsAs1DForOutWhenUnconnected=off
  S_DCDC : Outport  Port=2  VectorParamsAs1DForOutWhenUnconnected=off
  o_Idc : Outport  Port=3
  o_Ibat : Outport  Port=4
  o_Ilim : Outport  Port=5
  tag scope: Idc_f=global, Vdc_m=global, Vdc_ref=global, rpm_ref=global
  wires:
  iabc/1 -> RT_iabc/1
  Vdc filter/1 -> Sum1/2, [Vdc_m]
  Idc_max/1 -> Idc filter/1
  Abs_iabc/1 -> Idc_max/1
  Vref_min/1 -> Sum1/1
  RT_iabc/1 -> Abs_iabc/1
  Ibat_est/1 -> o_Ibat/1
  I_sq_minus/1 -> I2t_budget/1
  Idc filter/1 -> Ibat_est/1, [Idc_f], I_sq/2, I_sq/1, Ierr/2, o_Idc/1
  I_sq/1 -> I_sq_minus/1
  Vdc/1 -> Rate Transition2/1
  I_cont_sq/1 -> I_sq_minus/2
  Lim_sat/1 -> Vref_min/2
  Ierr/1 -> Lim_Kp/1, Lim_Ki/1
  I_cont_c/1 -> Ilim_switch/1
  I2t_budget/1 -> Ilim_switch/2
  Hall/1 -> Rate Transition4/1
  I_peak_c/1 -> Ilim_switch/3
  Ilim_switch/1 -> Ierr/1, o_Ilim/1
  RPMReq/1 -> Rate Transition6/1
  rpm/1 -> Rate Transition1/1
  Constant/1 -> Speed controller/2
  Rate Transition6/1 -> Abs/1, Sign/1(u), [rpm_ref]
  Sum1/1 -> Voltage controller/1
  Sum/1 -> Speed controller/1
  Rate Transition1/1 -> Product/1
  Rate Transition2/1 -> Vdc filter/1
  Sign/1(y) -> Product/2, Commutation/1(dir)
  Lim_Ki/1 -> Lim_Iint/1
  Rate Transition4/1 -> Commutation/2(Hall)
  Abs/1 -> Sum/1
  Constant1/1 -> Voltage controller/2
  Product/1 -> Sum/2
  Lim_Kp/1 -> Lim_PI_sum/1
  Lim_Iint/1 -> Lim_PI_sum/2
  Commutation/1(S) -> Rate Transition3/1
  Lim_PI_sum/1 -> Lim_sat/1
  Rate Transition3/1 -> S/1
  Speed controller/1 -> Vref_min/1, [Vdc_ref]
  Voltage controller/1 -> PWM/1(DC), Ibat_est/2
  PWM/1(G1) -> S_DCDC/1

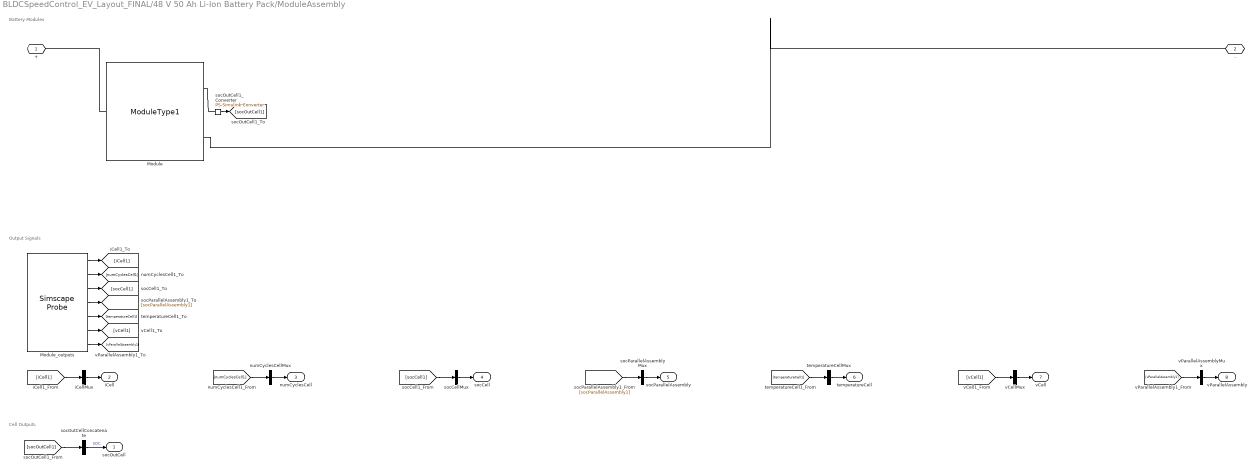
== system BLDCSpeedControl_EV_Layout_FINAL/48 V 50 Ah Li-Ion Battery Pack/ModuleAssembly ==
  note: Battery Modules
  note: Output Signals
  note: Cell Outputs
  Module : Batteries2_lib/Modules/ModuleType1  SOC_vecCell=[0, .1, .25, .5, .75, .9, 1]  SOC_vecCellPercentDeviation=zeros([130, 1])  T_vecCell=[278, 293, 313] K  T_vecCellPercentDeviation=zeros([130, 1])  V0_matCell=[3.49, 3.5, 3.51; 3.55, 3.57, 3.56; 3.62, 3.63, 3.64; 3.71, 3.71, 3.72; 3.91, 3.93, 3.94; 4.07, 4.08, 4.08; 4.19, 4.19, 4.19] V  V0_matCellPercentDeviation=zeros([130, 1])  V_rangeCell=[0, inf] V  V_rangeCellPercentDeviation=zeros([130, 1])  R0_matCell=[.0117, .0085, .009; .011, .0085, .009; .0114, .0087, .0092; .0107, .0082, .0088; .0107, .0083, .0091; .0113, .0085, .0089; .0116, .0085, .0089] Ohm  R0_matCellPercentDeviation=zeros([130, 1])  AHCell=5 A*hr  AHCellPercentDeviation=zeros([130, 1])  extrapolation_optionCell=simscape.enum.extrapolation.nearest  thermal_massCell=100 J/K  thermal_massCellPercentDeviation=zeros([130, 1])  P=10  S=13  iCell_specify=off  iCell_priority=None  iCell=repmat(0, 130, 1) A  iCell_nominal_specify=off  iCell_nominal_value=1  iCell_nominal_unit=A  vCell_specify=off  vCell_priority=None  vCell=repmat(0, 130, 1) V  vCell_nominal_specify=off  vCell_nominal_value=1  vCell_nominal_unit=V  socCell_specify=off  socCell_priority=High  socCell=repmat(1, 130, 1)  socCell_nominal_specify=off  socCell_nominal_value=1  socCell_nominal_unit=1  numCyclesCell_specify=off  numCyclesCell_priority=High  numCyclesCell=repmat(0, 130, 1)  numCyclesCell_nominal_specify=off  numCyclesCell_nominal_value=1  numCyclesCell_nominal_unit=1  temperatureCell_specify=off  temperatureCell_priority=High  temperatureCell=repmat(298.15, 130, 1) K  temperatureCell_nominal_specify=off  temperatureCell_nominal_value=1  temperatureCell_nominal_unit=K  vParallelAssembly_specify=off  vParallelAssembly_priority=None  vParallelAssembly=repmat(0, 13, 1) V  vParallelAssembly_nominal_specify=off  vParallelAssembly_nominal_value=1  vParallelAssembly_nominal_unit=V  socParallelAssembly_specify=off  socParallelAssembly_priority=None  socParallelAssembly=repmat(1, 13, 1)  socParallelAssembly_nominal_specify=off  socParallelAssembly_nominal_value=1  socParallelAssembly_nominal_unit=1
      settings: InternalSimscapePortConfiguration="{\"Bottom\":[{\"id\":\"n\",\"label\":\"-\",\"type\":\"foundation.electrical.electrical\"}],\"Left\":[],\"Right\":[{\"id\":\"socOutCell\",\"label\":\"SOC\",\"type\":\"output\"}],\"Top\":[{\"id\":\"p\",\"label\":\"+\",\"type\":\"foundation.electrical.electrical\"}]}"
  Module_outputs : SimscapeProbe  BoundBlock=1416  Variables="{\"iCell\":{\"Unit\":\"A\",\"PortLabel\":\"iCell\",\"Probing\":\"ON\"},\"numCyclesCell\":{\"Unit\":\"1\",\"PortLabel\":\"numCyclesCell\",\"Probing\":\"ON\"},\"socCell\":{\"Unit\":\"1\",\"PortLabel\":\"socCell\",\"Probing\":\"ON\"},\"socParallelAssembly\":{\"Unit\":\"1\",\"PortLabel\":\"socParallelAssembly\",\"Probing\":\"ON\"},\"temperatureCell\":{\"Unit\":\"K\",\"PortLabel\":\"temperatureCell\",\"Probing\":\"ON\"},\"vCell\":{\"Unit\":\"V\",\"PortLabel\":\"vCell\",\"Probing\":\"ON\"},\"vParallelAssembly\":{\"Unit\":\"V\",\"PortLabel\":\"vParallelAssembly\",\"Probing\":\"ON\"}}"
  iCellMux : Mux  Inputs=1
  numCyclesCellMux : Mux  Inputs=1
  socCellMux : Mux  Inputs=1
  socOutCell1_Converter : nesl_utility/PS-Simulink Converter  PhysicalDomain=network_engine_domain  SubClassName=ps_output  LeftPortType=input  RightPortType=output  PseudoPeriodic=off  Frequencies=[]  VectorFormat=inherit  Unit=inherit  AffineConversion=off
  socOutCellConcatenate : Concatenate  NumInputs=1  Mode=Multidimensional array  ConcatenateDimension=2
  socParallelAssemblyMux : Mux  Inputs=1
  temperatureCellMux : Mux  Inputs=1
  vCellMux : Mux  Inputs=1
  vParallelAssemblyMux : Mux  Inputs=1
  + : PMIOPort  Side=Left
  - : PMIOPort  Port=2  Side=Right
  socOutCell : Outport
  iCell : Outport  Port=2
  numCyclesCell : Outport  Port=3
  socCell : Outport  Port=4
  socParallelAssembly : Outport  Port=5
  temperatureCell : Outport  Port=6
  vCell : Outport  Port=7
  vParallelAssembly : Outport  Port=8
  wires:
  socOutCellConcatenate/1 -> socOutCell/1  "SOC"
  [socOutCell1] -> socOutCellConcatenate/1
  Module_outputs/1 -> [iCell1]
  iCellMux/1 -> iCell/1
  [iCell1] -> iCellMux/1
  Module_outputs/2 -> [numCyclesCell1]
  numCyclesCellMux/1 -> numCyclesCell/1
  [numCyclesCell1] -> numCyclesCellMux/1
  Module_outputs/3 -> [socCell1]
  socCellMux/1 -> socCell/1
  [socCell1] -> socCellMux/1
  Module_outputs/4 -> [socParallelAssembly1]
  socParallelAssemblyMux/1 -> socParallelAssembly/1
  [socParallelAssembly1] -> socParallelAssemblyMux/1
  Module_outputs/5 -> [temperatureCell1]
  temperatureCellMux/1 -> temperatureCell/1
  [temperatureCell1] -> temperatureCellMux/1
  Module_outputs/6 -> [vCell1]
  vCellMux/1 -> vCell/1
  [vCell1] -> vCellMux/1
  Module_outputs/7 -> [vParallelAssembly1]
  vParallelAssemblyMux/1 -> vParallelAssembly/1
  [vParallelAssembly1] -> vParallelAssemblyMux/1
  socOutCell1_Converter/1 -> [socOutCell1]
  connections:
  Module/LConn1 -- +/RConn1
  Module/RConn2 -- -/RConn1
  socOutCell1_Converter/LConn1 -- Module/RConn1

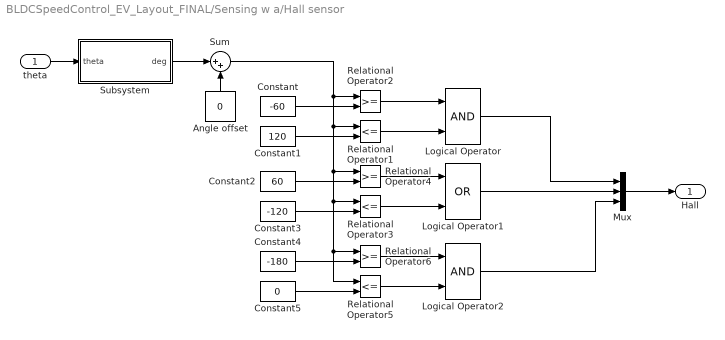
== system BLDCSpeedControl_EV_Layout_FINAL/Sensing w a/Hall sensor ==
  theta : Inport
  Angle offset : Constant  Value=0
  Constant : Constant  Value=-60
  Constant1 : Constant  Value=120
  Constant2 : Constant  Value=60
  Constant3 : Constant  Value=-120
  Constant4 : Constant  Value=-180
  Constant5 : Constant  Value=0
  Logical Operator : Logic  AllPortsSameDT=off  OutDataTypeStr=boolean
  Logical Operator1 : Logic  Operator=OR  AllPortsSameDT=off  OutDataTypeStr=boolean
  Logical Operator2 : Logic  AllPortsSameDT=off  OutDataTypeStr=boolean
  Mux : Mux  Inputs=3
  Relational Operator1 : RelationalOperator  Operator=<=
  Relational Operator2 : RelationalOperator
  Relational Operator3 : RelationalOperator  Operator=<=
  Relational Operator4 : RelationalOperator
  Relational Operator5 : RelationalOperator  Operator=<=
  Relational Operator6 : RelationalOperator
  Subsystem : Subsystem
  Sum : Sum  Inputs=|++
  Hall : Outport  VectorParamsAs1DForOutWhenUnconnected=off
  wires:
  Constant3/1 -> Relational Operator3/2
  Logical Operator2/1 -> Mux/3
  Logical Operator1/1 -> Mux/2
  Logical Operator/1 -> Mux/1
  Relational Operator5/1 -> Logical Operator2/2
  Relational Operator6/1 -> Logical Operator2/1
  Constant4/1 -> Relational Operator6/2
  Constant5/1 -> Relational Operator5/2
  Relational Operator3/1 -> Logical Operator1/2
  Mux/1 -> Hall/1
  Relational Operator2/1 -> Logical Operator/1
  Relational Operator1/1 -> Logical Operator/2
  Constant/1 -> Relational Operator2/2
  Relational Operator4/1 -> Logical Operator1/1
  Constant1/1 -> Relational Operator1/2
  Constant2/1 -> Relational Operator4/2
  theta/1 -> Subsystem/1(theta)
  Subsystem/1(deg) -> Sum/1
  Sum/1 -> Relational Operator1/1, Relational Operator5/1, Relational Operator6/1, Relational Operator3/1, Relational Operator4/1, Relational Operator2/1
  Angle offset/1 -> Sum/2

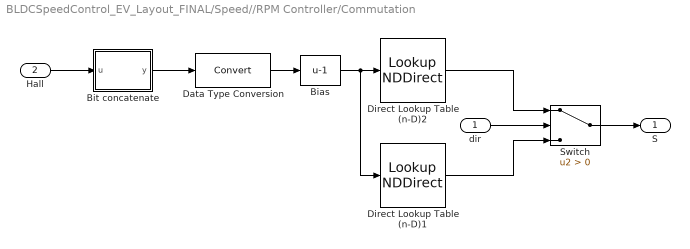
== system BLDCSpeedControl_EV_Layout_FINAL/Speed//RPM Controller/Commutation ==
  dir : Inport
  Hall : Inport  Port=2
  Bias : Bias  Bias=-1  SaturateOnIntegerOverflow=off
  Bit concatenate : Subsystem
  Data Type Conversion : DataTypeConversion  SaturateOnIntegerOverflow=off  RndMeth=Floor
  Direct Lookup Table (n-D)1 : LookupNDDirect  InputsSelectThisObjectFromTable=Vector  Table=[0 1 1 0 0 0;0 0 0 1 1 0;1 0 0 0 1 0;0 1 0 0 0 1;0 0 0 1 0 1;1 0 1 0 0 0]
  Direct Lookup Table (n-D)2 : LookupNDDirect  InputsSelectThisObjectFromTable=Vector  Table=[0 0 0 1 1 0;0 1 1 0 0 0;0 1 0 0 0 1;1 0 0 0 1 0;1 0 1 0 0 0;0 0 0 1 0 1]
  Switch : Switch  Criteria=u2 > Threshold  SaturateOnIntegerOverflow=off  InputSameDT=off
  S : Outport  VectorParamsAs1DForOutWhenUnconnected=off
  wires:
  Hall/1 -> Bit concatenate/1(u)
  Bit concatenate/1(y) -> Data Type Conversion/1
  Data Type Conversion/1 -> Bias/1
  Bias/1 -> Direct Lookup Table (n-D)1/1, Direct Lookup Table (n-D)2/1
  Switch/1 -> S/1
  dir/1 -> Switch/2
  Direct Lookup Table (n-D)2/1 -> Switch/1
  Direct Lookup Table (n-D)1/1 -> Switch/3

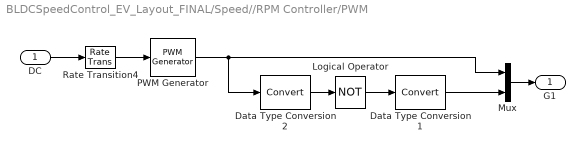
== system BLDCSpeedControl_EV_Layout_FINAL/Speed//RPM Controller/PWM ==
  DC : Inport
  Data Type Conversion1 : DataTypeConversion  SaturateOnIntegerOverflow=off  RndMeth=Floor
  Data Type Conversion2 : DataTypeConversion  SaturateOnIntegerOverflow=off  RndMeth=Floor
  Logical Operator : Logic  Operator=NOT  AllPortsSameDT=off  OutDataTypeStr=boolean
  Mux : Mux  Inputs=2
  PWM Generator : eePwmGenerator/PWM Generator  CarrCount=Up  Tper=Tsc  Tdelay=0  Ts=Ts
  Rate Transition4 : RateTransition  OutPortSampleTime=Ts
  G1 : Outport  VectorParamsAs1DForOutWhenUnconnected=off
  wires:
  Mux/1 -> G1/1
  Rate Transition4/1 -> PWM Generator/1
  PWM Generator/1 -> Data Type Conversion2/1, Mux/1
  Data Type Conversion1/1 -> Mux/2
  Logical Operator/1 -> Data Type Conversion1/1
  DC/1 -> Rate Transition4/1
  Data Type Conversion2/1 -> Logical Operator/1

== system BLDCSpeedControl_EV_Layout_FINAL/Speed//RPM Controller/Sign ==
  u : Inport
  Constant2 : Constant
  Constant3 : Constant  Value=-1
  Switch : Switch  SaturateOnIntegerOverflow=off  InputSameDT=off
  y : Outport
  wires:
  Constant3/1 -> Switch/3
  Constant2/1 -> Switch/1
  u/1 -> Switch/2
  Switch/1 -> y/1
